simulink subsystem "Telescoping_Tube"  (R2024b)
settings: Solver=VariableStepAuto  StartTime=0.0  StopTime=10.0  RelTol=1e-3
model mask{i=1}
  mask prompts: i "Tube No."
values from neighbouring files (symbols this model uses):
  L = [650, 640, 640, 640, 640, 640, 640, 640,       640, 640, 640, 640, 640, 640, 600, 600]    [print_properties.m]    (also in single_tube_deflection.m = 0.64)
  m = [227.7, 160.8, 155.0, 152.0, 138.9, 130.6, 123.3, 114.7,        99.5,  93.2,  84.7,  75.5,  67.4,  59.2,  45.0,  38.6]    [print_properties.m]
  X = R .* cos(PHI + theta) + x    [single_tube_deflection.m]
  Y = R .* sin(PHI + theta)    [single_tube_deflection.m]
  Z = ones(size(X)) * z    [single_tube_deflection.m]
undefined symbols (not defined in the file or in its folder): d_i, d_o
libraries: sm_lib x4, nesl_utility x3
settings Model: Creator=brice  LastModifiedBy=brice

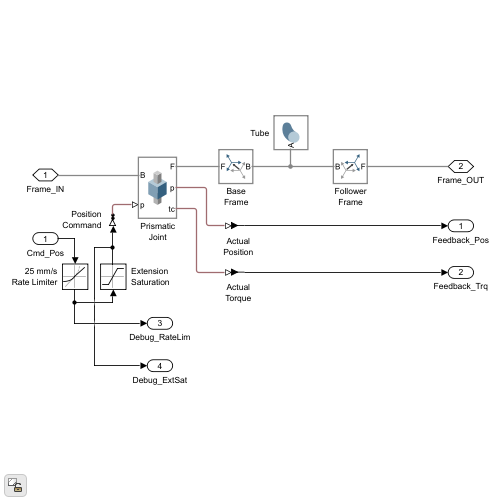
[thumbnail: Simulink's stored preview of the top-level diagram]
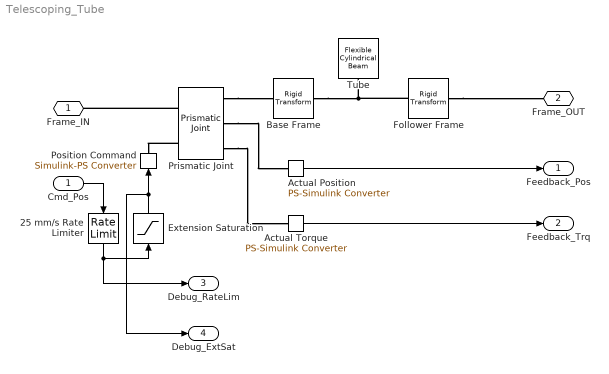
== system Telescoping_Tube ==
  Cmd_Pos : Inport
  25 mm/s Rate Limiter : RateLimiter  RisingSlewLimit=25  FallingSlewLimit=-25  SampleTimeMode=inherited
  Actual Position : nesl_utility/PS-Simulink Converter  PhysicalDomain=network_engine_domain  SubClassName=ps_output  LeftPortType=input  RightPortType=output  PseudoPeriodic=off  Frequencies=[]  VectorFormat=inherit  Unit=mm  AffineConversion=off
  Actual Torque : nesl_utility/PS-Simulink Converter  PhysicalDomain=network_engine_domain  SubClassName=ps_output  LeftPortType=input  RightPortType=output  PseudoPeriodic=off  Frequencies=[]  VectorFormat=inherit  Unit=inherit  AffineConversion=off
  Base Frame : sm_lib/Frames and Transforms/Rigid Transform  RotationMethod=None  FollAlignAxisA=+X  BaseAlignAxisA=+Y  FollAlignAxisB=+Y  BaseAlignAxisB=+Z  RotationStandardAxis=+Z  RotationAngle=0.0  RotationAngleUnits=deg  RotationArbitraryAxis=[0 0 1]  RotationSequenceAxes=FollowerAxes  RotationSequence=XYX  RotationSequenceAngles=[0 0 0]  RotationSequenceAnglesUnits=deg  RotationMatrix=[1 0 0; 0 1 0; 0 0 1]  Quaternion=[1 0 0 0]  TranslationMethod=StandardAxis  TranslationCartesianOffset=[0 0 0]  TranslationCartesianOffsetUnits=m  TranslationStandardAxis=-Z  TranslationStandardOffset=0  TranslationStandardOffsetUnits=mm  TranslationROffset=0  TranslationROffsetUnits=m  TranslationThetaOffset=0  TranslationThetaOffsetUnits=deg  TranslationZOffset=0  TranslationZOffsetUnits=m
  Extension Saturation : Saturate  UpperLimit=L(i)-150  LowerLimit=0  OutDataTypeStr=Inherit: Inherit via back propagation
  Follower Frame : sm_lib/Frames and Transforms/Rigid Transform  RotationMethod=None  FollAlignAxisA=+X  BaseAlignAxisA=+Y  FollAlignAxisB=+Y  BaseAlignAxisB=+Z  RotationStandardAxis=+Z  RotationAngle=0.0  RotationAngleUnits=deg  RotationArbitraryAxis=[0 0 1]  RotationSequenceAxes=FollowerAxes  RotationSequence=XYX  RotationSequenceAngles=[0 0 0]  RotationSequenceAnglesUnits=deg  RotationMatrix=[1 0 0; 0 1 0; 0 0 1]  Quaternion=[1 0 0 0]  TranslationMethod=StandardAxis  TranslationCartesianOffset=[0 0 0]  TranslationCartesianOffsetUnits=m  TranslationStandardAxis=+Z  TranslationStandardOffset=0  TranslationStandardOffsetUnits=mm  TranslationROffset=0  TranslationROffsetUnits=m  TranslationThetaOffset=0  TranslationThetaOffsetUnits=deg  TranslationZOffset=0  TranslationZOffsetUnits=m
  Position Command : nesl_utility/Simulink-PS Converter  PhysicalDomain=network_engine_domain  SubClassName=ps_input  LeftPortType=input  RightPortType=output  PseudoPeriodic=off  Frequencies=[]  NoiseDistribution=none  NoiseParameters=[]  Unit=mm  AffineConversion=off  FilteringAndDerivatives=filter  SimscapeFilterOrder=2  InputFilterTimeConstant=0.001  UdotUserProvided=0
  Prismatic Joint : sm_lib/Joints/Prismatic Joint  JointMode=Normal  CompositeWrenchDir=BaseOnFollower  CompositeWrenchFrame=BaseFrame  SenseConstraintForce=off  SenseConstraintTorque=on  SenseTotalForce=off  SenseTotalTorque=off  PositionTargetSpecify=on  PositionTargetPriority=High  PositionTargetValue=0  PositionTargetValueUnits=mm  VelocityTargetSpecify=on  VelocityTargetPriority=High  VelocityTargetValue=0  VelocityTargetValueUnits=mm/s  EquilibriumPosition=0  EquilibriumPositionUnits=m  SpringStiffness=0  SpringStiffnessUnits=N/m  DampingCoefficient=0  DampingCoefficientUnits=N/(m/s)  LowerLimitSpecify=on  LowerLimitBound=0  LowerLimitBoundUnits=mm  LowerLimitStiffness=1e6  LowerLimitStiffnessUnits=N/m  LowerLimitDamping=1e5  LowerLimitDampingUnits=N/(m/s)  LowerLimitTransitionRegionWidth=1  LowerLimitTransitionRegionWidthUnits=mm  UpperLimitSpecify=on  UpperLimitBound=L(i)-150  UpperLimitBoundUnits=mm  UpperLimitStiffness=1e6  UpperLimitStiffnessUnits=N/m  UpperLimitDamping=1e5  UpperLimitDampingUnits=N/(m/s)  UpperLimitTransitionRegionWidth=1  UpperLimitTransitionRegionWidthUnits=mm  TorqueActuationMode=ComputedTorque  MotionActuationMode=InputMotion  SensePosition=on  SenseVelocity=off  SenseAcceleration=off  SenseTorqueForce=off  SenseLowerLimitTorqueForce=off  SenseUpperLimitTorqueForce=off
  Tube : sm_lib/Body Elements/Flexible Bodies/Beams/Flexible Cylindrical Beam  SectionType=Hollow  Radius=d_o(i)/2  RadiusUnits=mm  Thickness=(d_o(i) - d_i(i))/2  ThicknessUnits=mm  Length=L(i)  LengthUnits=mm  StiffnessAndInertiaType=CalculateFromGeometry  Density=rho_gfrp  DensityUnits=kg/m^3  ModuliType=YoungsShear  YoungsModulus=E_gfrp  YoungsModulusUnits=GPa  PoissonsRatio=0.33  ShearModulus=G_gfrp  ShearModulusUnits=GPa  GeometricCentroid=[0 0]  GeometricCentroidUnits=m  BendingCentroid=[0 0]  BendingCentroidUnits=m  ShearCenter=[0 0]  ShearCenterUnits=m  AxialRigidity=1  AxialRigidityUnits=Pa*m^2  FlexuralRigidity=[1 1]  FlexuralRigidityUnits=Pa*m^4  CrossFlexuralRigidity=0  CrossFlexuralRigidityUnits=Pa*m^4  TorsionalRigidity=1  TorsionalRigidityUnits=Pa*m^4  CenterOfMass=[0 0]  CenterOfMassUnits=m  MassPerUnitLength=1  MassPerUnitLengthUnits=kg/m  MassMomentOfInertiaDensity=[1 1]  MassMomentOfInertiaDensityUnits=kg*m  MassProductOfInertiaDensity=0  MassProductOfInertiaDensityUnits=kg*m  DampingType=Proportional  ProportionalDampingAlpha=0  ProportionalDampingAlphaUnits=1/s  ProportionalDampingBeta=0.001  ProportionalDampingBetaUnits=s  UniformModalDampingRatio=0.01  NumElements=1  ReductionType=None  NumRetainedModes=1  GraphicType=FromGeometry  GraphicVisPropType=SimpleVisualProperties  GraphicDiffuseColor=[1 0 0]  GraphicOpacity=1  GraphicSpecularColor=[0.5 0.5 0.5 1.0]  GraphicAmbientColor=[0.15 0.15 0.15 1.0]  GraphicEmissiveColor=[0.0 0.0 0.0 1.0]  GraphicShininess=75  DoExposeZminFrame=on  DoExposeZmaxFrame=off  SerializedFrames=<Frames/>
  Frame_IN : PMIOPort  Side=Left
  Frame_OUT : PMIOPort  Port=2  Side=Right
  Feedback_Pos : Outport
  Feedback_Trq : Outport  Port=2
  Debug_RateLim : Outport  Port=3
  Debug_ExtSat : Outport  Port=4
  wires:
  Actual Torque/1 -> Feedback_Trq/1
  Actual Position/1 -> Feedback_Pos/1
  25 mm/s Rate Limiter/1 -> Extension Saturation/1, Debug_RateLim/1
  Cmd_Pos/1 -> 25 mm/s Rate Limiter/1
  Extension Saturation/1 -> Position Command/1, Debug_ExtSat/1
  connections:
  Base Frame/LConn1 -- Follower Frame/LConn1 -- Tube/LConn1
  Prismatic Joint/RConn3 -- Actual Torque/LConn1
  Prismatic Joint/RConn1 -- Base Frame/RConn1
  Prismatic Joint/RConn2 -- Actual Position/LConn1
  Prismatic Joint/LConn1 -- Frame_IN/RConn1
  Follower Frame/RConn1 -- Frame_OUT/RConn1
  Prismatic Joint/LConn2 -- Position Command/RConn1
